simulink model "NIBB_TwoStage"  (R2022a)
settings: Solver=ode23tb  StartTime=0.0  StopTime=0.35  FixedStep=2e-7  MaxStep=2e-7  RelTol=1e-3
libraries: spsSeriesRLCBranchLib x6, simulink x3, spsDiodeLib x3, spsMosfetLib x3, spsVoltageMeasurementLib x3, spsCurrentMeasurementLib x2, spsMeanLib x2, eePowerMeasurement x2, spsDCVoltageSourceLib x1, spsMultimeterLib x1, spspowerguiLib x1
settings Model: SimulationMode=accelerator  Creator=Bobby  LastModifiedBy=Bobby

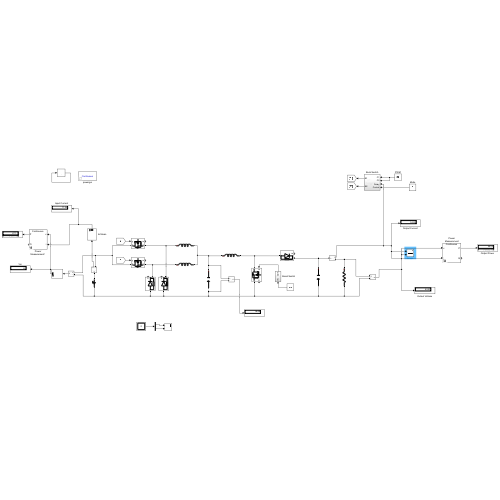
[thumbnail: Simulink's stored preview of the top-level diagram]
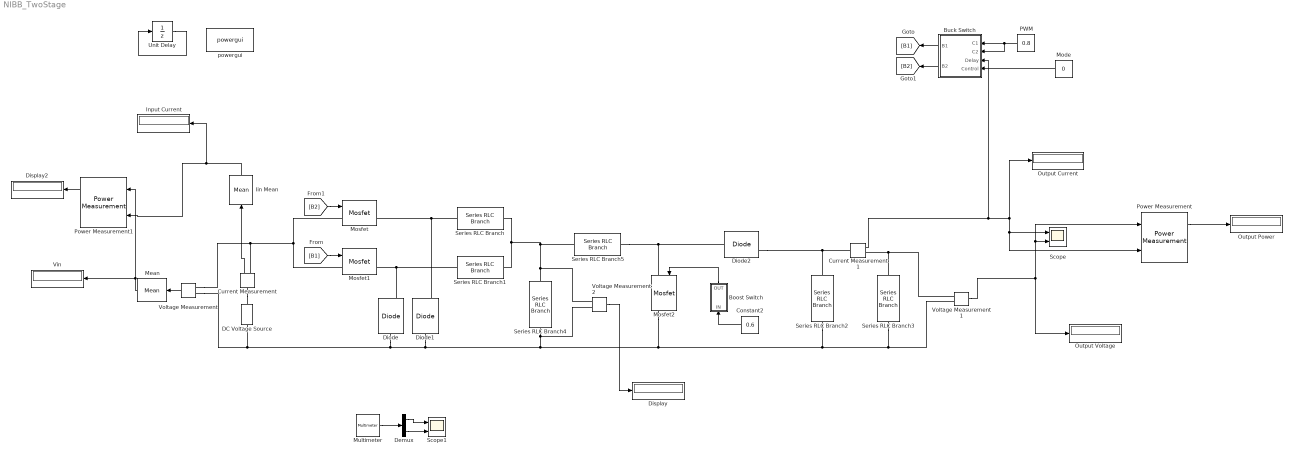
== system NIBB_TwoStage ==
  Boost Switch : Subsystem
  Buck Switch : Subsystem
  Constant2 : Constant  Value=0.6
  Current Measurement : spsCurrentMeasurementLib/Current Measurement  PhasorSimulation=off  OutputType=Complex  PSBequivalent=0
  Current Measurement1 : spsCurrentMeasurementLib/Current Measurement  PhasorSimulation=off  OutputType=Complex  PSBequivalent=0
  DC Voltage Source : spsDCVoltageSourceLib/DC Voltage Source  Amplitude=24  Measurements=None
  Demux : Demux  Outputs=2
  Diode : spsDiodeLib/Diode  Ron=0.001  Lon=0  Vf=0.8  IC=0  UseSnubber=0  Rs=500  Cs=250e-9  Measurements=on
  Diode1 : spsDiodeLib/Diode  Ron=0.001  Lon=0  Vf=0.8  IC=0  UseSnubber=0  Rs=500  Cs=250e-9  Measurements=on
  Diode2 : spsDiodeLib/Diode  Ron=0.001  Lon=0  Vf=0.8  IC=0  UseSnubber=0  Rs=500  Cs=250e-9  Measurements=on
  Display : Display
  Display2 : Display
  Iin Mean : spsMeanLib/Mean  Freq=60  Vinit=0  Ts=0
  Input Current : Display
  Mean : spsMeanLib/Mean  Freq=60  Vinit=0  Ts=0
  Mode : Constant  Value=0
  Mosfet : spsMosfetLib/Mosfet  Ron=0.1  Lon=0  Rd=0.01  Vfd=0  IC=0  Rs=1e5  Cs=inf  Measurements=on
  Mosfet1 : spsMosfetLib/Mosfet  Ron=0.1  Lon=0  Rd=0.01  Vfd=0  IC=0  Rs=1e5  Cs=inf  Measurements=on
  Mosfet2 : spsMosfetLib/Mosfet  Ron=0.1  Lon=0  Rd=0.01  Vfd=0  IC=0  Rs=1e5  Cs=inf  Measurements=on
  Multimeter : spsMultimeterLib/Multimeter  L=3  sel=[1 2]  yselected={}  Gain=[1 1]  OutputType=Complex  PlotAtSimulationStop=off  PhasorSimulation=off
  Output Current : Display
  Output Power : Display
  Output Voltage : Display
  PWM : Constant  Value=0.8
  Power Measurement : eePowerMeasurement/Power Measurement  LabelModeActiveChoice=Continuous  F=60  K=[0 1 2 3]  Ts=0
      settings: SourceProductBaseCode=PS
  Power Measurement1 : eePowerMeasurement/Power Measurement  LabelModeActiveChoice=Continuous  F=60  K=[0 1 2 3]  Ts=0
      settings: SourceProductBaseCode=PS
  Scope : Scope  NumInputPorts=2
  Scope1 : Scope  NumInputPorts=2
  Series RLC Branch : spsSeriesRLCBranchLib/Series RLC Branch  LConnTagsString=__new0  RConnTagsString=__new0  BranchType=L  Resistance=1  Inductance=80e-6  SetiL0=off  InitialCurrent=0  Capacitance=1e-6  Setx0=off  InitialVoltage=0  Measurements=Branch current
  Series RLC Branch1 : spsSeriesRLCBranchLib/Series RLC Branch  LConnTagsString=__new0  RConnTagsString=__new0  BranchType=L  Resistance=1  Inductance=80e-6  SetiL0=off  InitialCurrent=0  Capacitance=1e-6  Setx0=off  InitialVoltage=0  Measurements=Branch current
  Series RLC Branch2 : spsSeriesRLCBranchLib/Series RLC Branch  LConnTagsString=__new0  RConnTagsString=__new0  BranchType=C  Resistance=1  Inductance=1e-3  SetiL0=off  InitialCurrent=0  Capacitance=1666e-6  Setx0=off  InitialVoltage=0  Measurements=None
  Series RLC Branch3 : spsSeriesRLCBranchLib/Series RLC Branch  LConnTagsString=__new0  RConnTagsString=__new0  BranchType=R  Resistance=7.68  Inductance=1e-3  SetiL0=off  InitialCurrent=0  Capacitance=1e-6  Setx0=off  InitialVoltage=0  Measurements=None
  Series RLC Branch4 : spsSeriesRLCBranchLib/Series RLC Branch  LConnTagsString=__new0  RConnTagsString=__new0  BranchType=C  Resistance=1  Inductance=1e-3  SetiL0=off  InitialCurrent=0  Capacitance=150e-6  Setx0=off  InitialVoltage=0  Measurements=None
  Series RLC Branch5 : spsSeriesRLCBranchLib/Series RLC Branch  LConnTagsString=__new0  RConnTagsString=__new0  BranchType=L  Resistance=1  Inductance=80e-6  SetiL0=off  InitialCurrent=0  Capacitance=1e-6  Setx0=off  InitialVoltage=0  Measurements=Branch current
  Unit Delay : UnitDelay  SampleTime=-1  HasFrameUpgradeWarning=on
  Vin : Display
  Voltage Measurement : spsVoltageMeasurementLib/Voltage Measurement  PhasorSimulation=off  OutputType=Complex  PSBequivalent=0
  Voltage Measurement1 : spsVoltageMeasurementLib/Voltage Measurement  PhasorSimulation=off  OutputType=Complex  PSBequivalent=0
  Voltage Measurement2 : spsVoltageMeasurementLib/Voltage Measurement  PhasorSimulation=off  OutputType=Complex  PSBequivalent=0
  powergui : spspowerguiLib/powergui  Priority=1  SimulationMode=Continuous  SampleTime=50e-6  frequency=60  Iterations=50  frequencyindice=0  Pbase=100e6  ErrMax=1e-4  UnitsV=kV  UnitsW=MW  buscounter=0  FunctionMessages=off  echomessages=off  EnableUseOfTLC=off  CurrentSourceSwitches=off  DisableSnubberDevices=off  DisableRonSwitches=off  DisableVfSwitches=off  DisplayEquations=off  AutomaticDiscreteSolvers=off  SolverType=Tustin/Backward Euler (TBE)  Interpol=off  ExternalGateDelay=off  methode=off  Ts=100  x0status=blocks  SPID=on  SwTol=0  HookPort=off  NonlinearTolerance=1e-4  nMaxIteration=100  ContinueOnMaxIteration=off  RestoreLinks=warning  ResistiveCurrentMeasurement=off  Frange=[0:2:500]  Ylog=off  Xlog=on  ShowGrid=off  save=off  variable=ZData  structure=0  ZoomFFT=off  StartTime=0.0  cycles=1  DisplayStyle=1  fundamental=60  FreqAxis=off  MaxFrequency=1000  frequencyindicesteady=1  RmsSteady=1  display=off
  wires:
  Current Measurement1/1 -> Buck Switch/3(Delay), Power Measurement/2, Scope/1, Output Current/1
  Voltage Measurement1/1 -> Power Measurement/1, Scope/2, Output Voltage/1
  Power Measurement/1 -> Output Power/1
  Voltage Measurement/1 -> Mean/1
  Current Measurement/1 -> Iin Mean/1
  Mean/1 -> Vin/1, Power Measurement1/1
  Iin Mean/1 -> Input Current/1, Power Measurement1/2
  Power Measurement1/1 -> Display2/1
  Unit Delay/1 -> Unit Delay/1
  Multimeter/1 -> Demux/1
  Demux/2 -> Scope1/2
  Demux/1 -> Scope1/1
  Constant2/1 -> Boost Switch/1("IN ")
  Boost Switch/1(OUT) -> Mosfet2/1
  PWM/1 -> Buck Switch/2(C2), Buck Switch/1(C1)
  [B1] -> Mosfet1/1
  [B2] -> Mosfet/1
  Buck Switch/1(B1) -> [B1]
  Buck Switch/2(B2) -> [B2]
  Mode/1 -> Buck Switch/4(Control)
  Voltage Measurement2/1 -> Display/1
  connections:
  Current Measurement/LConn1 -- DC Voltage Source/RConn1
  Current Measurement/RConn1 -- Voltage Measurement/LConn1 -- Mosfet/LConn1 -- Mosfet1/LConn1
  Diode/LConn1 -- Voltage Measurement2/LConn2 -- Series RLC Branch4/RConn1 -- Voltage Measurement1/LConn2 -- Series RLC Branch3/RConn1 -- Series RLC Branch2/RConn1 -- Mosfet2/RConn1 -- Diode1/LConn1 -- Voltage Measurement/LConn2 -- DC Voltage Source/LConn1
  Series RLC Branch/LConn1 -- Diode1/RConn1 -- Mosfet/RConn1
  Diode/RConn1 -- Series RLC Branch1/LConn1 -- Mosfet1/RConn1
  Diode2/RConn1 -- Current Measurement1/LConn1 -- Series RLC Branch2/LConn1
  Series RLC Branch3/LConn1 -- Voltage Measurement1/LConn1 -- Current Measurement1/RConn1
  Mosfet2/LConn1 -- Series RLC Branch5/RConn1 -- Diode2/LConn1
  Series RLC Branch/RConn1 -- Voltage Measurement2/LConn1 -- Series RLC Branch4/LConn1 -- Series RLC Branch5/LConn1 -- Series RLC Branch1/RConn1

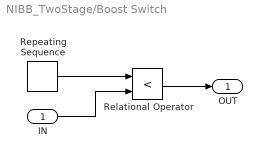
== system NIBB_TwoStage/Boost Switch ==
  "IN " : Inport
  Relational Operator : RelationalOperator  Operator=<  OutDataTypeStr=boolean  RndMeth=Simplest  InputSameDT=off
  Repeating Sequence : simulink/Sources/Repeating Sequence  rep_seq_t=[0, 1e-5, 2e-5]  rep_seq_y=[0 1 0]
  OUT : Outport
  wires:
  Repeating Sequence/1 -> Relational Operator/1
  "IN "/1 -> Relational Operator/2
  Relational Operator/1 -> OUT/1

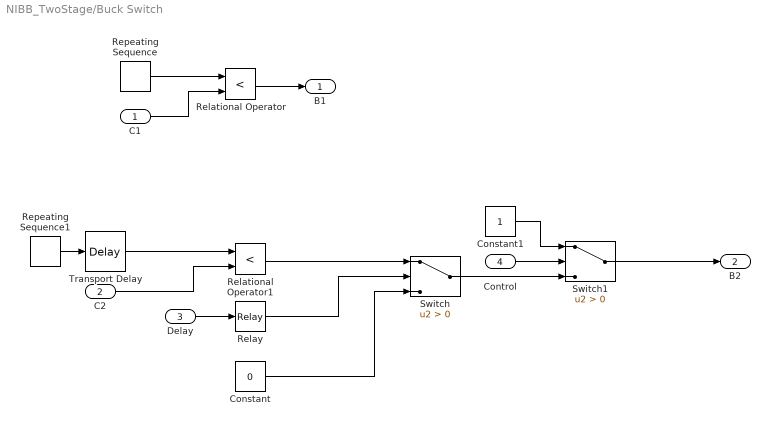
== system NIBB_TwoStage/Buck Switch ==
  C1 : Inport
  C2 : Inport  Port=2
  Delay : Inport  Port=3
  Control : Inport  Port=4
  Constant : Constant  Value=0
  Constant1 : Constant
  Relational Operator : RelationalOperator  Operator=<  OutDataTypeStr=boolean  RndMeth=Simplest  InputSameDT=off
  Relational Operator1 : RelationalOperator  Operator=<  OutDataTypeStr=boolean  RndMeth=Simplest  InputSameDT=off
  Relay : Relay  OnSwitchValue=2.5  OffSwitchValue=2.0
  Repeating Sequence : simulink/Sources/Repeating Sequence  rep_seq_t=[0, 1e-5, 2e-5]  rep_seq_y=[0 1 0]
  Repeating Sequence1 : simulink/Sources/Repeating Sequence  rep_seq_t=[0, 1e-5, 2e-5]  rep_seq_y=[0 1 0]
  Switch : Switch  Criteria=u2 > Threshold  SaturateOnIntegerOverflow=off  InputSameDT=off
  Switch1 : Switch  Criteria=u2 > Threshold  SaturateOnIntegerOverflow=off  InputSameDT=off
  Transport Delay : TransportDelay  DelayTime=1e-5
  B1 : Outport
  B2 : Outport  Port=2
  wires:
  Repeating Sequence/1 -> Relational Operator/1
  C1/1 -> Relational Operator/2
  Relational Operator/1 -> B1/1
  Repeating Sequence1/1 -> Transport Delay/1
  Transport Delay/1 -> Relational Operator1/1
  C2/1 -> Relational Operator1/2
  Relational Operator1/1 -> Switch/1
  Relay/1 -> Switch/2
  Constant/1 -> Switch/3
  Delay/1 -> Relay/1
  Switch1/1 -> B2/1
  Switch/1 -> Switch1/3
  Control/1 -> Switch1/2
  Constant1/1 -> Switch1/1
